simulink subsystem "fluxObserver"  (R2023b)
settings: Solver=VariableStepAuto  StartTime=0.0  StopTime=10.0  RelTol=1e-3
values from neighbouring files (symbols this model uses):
  motor = setMotorParameters("SynRelLaplace")    [initSimulinkObs.m]    (also in setMotorParameters.m = struct)
  Ts = 1e-4    (= 0.0001)    [initSimulinkObs.m]
undefined symbols (not defined in the file or in its folder): DiscIntNeverNeededParam, math, observer
settings Model: Creator=rdelpoux  LastModifiedBy=rdelpoux
settings ModelReferenceCC: UpdateModelReferenceTargets=IfOutOfDate
settings RTWCC: GPUComputeCapability=5.0
settings ConfigComp: CovBoundaryAbsTol=1.0e-5

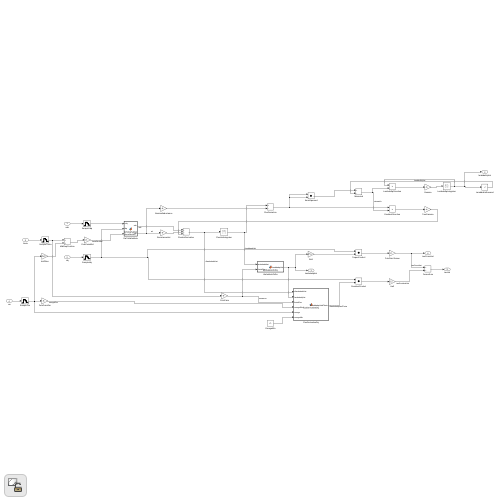
[thumbnail: Simulink's stored preview of the top-level diagram]
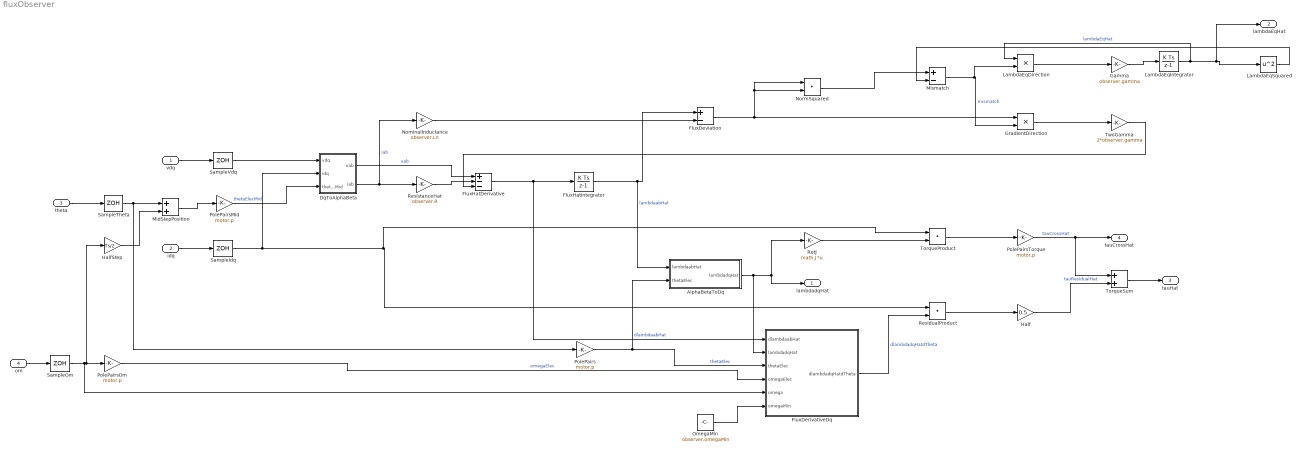
== system fluxObserver ==
  vdq : Inport
  idq : Inport  Port=2
  theta : Inport  Port=3
  om : Inport  Port=4
  AlphaBetaToDq : MATLAB Function  TreatAsAtomicUnit=on
  DqToAlphaBeta : MATLAB Function  TreatAsAtomicUnit=on
  FluxDerivativeDq : MATLAB Function  TreatAsAtomicUnit=on
  FluxDeviation : Sum  Inputs=+-
  FluxHatDerivative : Sum  Inputs=+--
  FluxHatIntegrator : DiscreteIntegrator  InitialCondition=observer.lambda0  SampleTime=Ts  ICPrevOutput=DiscIntNeverNeededParam  ICPrevScaledInput=DiscIntNeverNeededParam
  Gamma : Gain  Gain=observer.gamma
  GradientDirection : Product
  Half : Gain  Gain=0.5
  HalfStep : Gain  Gain=Ts/2
  LambdaEqDirection : Product
  LambdaEqIntegrator : DiscreteIntegrator  InitialCondition=observer.lambdaEq0  SampleTime=Ts  ICPrevOutput=DiscIntNeverNeededParam  ICPrevScaledInput=DiscIntNeverNeededParam
  LambdaEqSquared : Math  Operator=square
  MidStepPosition : Sum
  Mismatch : Sum  Inputs=+-
  NominalInductance : Gain  Gain=observer.Ln
  NormSquared : DotProduct  OutDataTypeStr=Inherit: Inherit via internal rule
  OmegaMin : Constant  Value=observer.omegaMin
  PolePairs : Gain  Gain=motor.p
  PolePairsMid : Gain  Gain=motor.p
  PolePairsOm : Gain  Gain=motor.p
  PolePairsTorque : Gain  Gain=motor.p
  ResidualProduct : DotProduct  OutDataTypeStr=Inherit: Inherit via internal rule
  ResistanceHat : Gain  Gain=observer.R
  RotJ : Gain  Gain=math.J  Multiplication=Matrix(K*u)
  SampleIdq : ZeroOrderHold  SampleTime=Ts
  SampleOm : ZeroOrderHold  SampleTime=Ts
  SampleTheta : ZeroOrderHold  SampleTime=Ts
  SampleVdq : ZeroOrderHold  SampleTime=Ts
  TorqueProduct : DotProduct  OutDataTypeStr=Inherit: Inherit via internal rule
  TorqueSum : Sum
  TwoGamma : Gain  Gain=2*observer.gamma
  lambdadqHat : Outport
  lambdaEqHat : Outport  Port=2
  tauHat : Outport  Port=3
  tauCrossHat : Outport  Port=4
  wires:
  PolePairsMid/1 -> DqToAlphaBeta/3(thetaElecMid)  "thetaElecMid"
  MidStepPosition/1 -> PolePairsMid/1
  HalfStep/1 -> MidStepPosition/2
  ResidualProduct/1 -> Half/1
  TorqueSum/1 -> tauHat/1
  Half/1 -> TorqueSum/2  "tauResidualHat"
  PolePairsTorque/1 -> tauCrossHat/1, TorqueSum/1  "tauCrossHat"
  SampleOm/1 -> FluxDerivativeDq/5(omega), HalfStep/1, PolePairsOm/1
  om/1 -> SampleOm/1
  AlphaBetaToDq/1(lambdadqHat) -> FluxDerivativeDq/2(lambdadqHat), RotJ/1, lambdadqHat/1
  TorqueProduct/1 -> PolePairsTorque/1
  RotJ/1 -> TorqueProduct/2
  Gamma/1 -> LambdaEqIntegrator/1
  LambdaEqDirection/1 -> Gamma/1
  FluxHatDerivative/1 -> FluxHatIntegrator/1, FluxDerivativeDq/1(dlambdaabHat)  "dlambdaabHat"
  TwoGamma/1 -> FluxHatDerivative/3
  ResistanceHat/1 -> FluxHatDerivative/2
  DqToAlphaBeta/1(vab) -> FluxHatDerivative/1  "vab"
  GradientDirection/1 -> TwoGamma/1
  Mismatch/1 -> LambdaEqDirection/2, GradientDirection/2  "mismatch"
  LambdaEqSquared/1 -> Mismatch/2
  NormSquared/1 -> Mismatch/1
  LambdaEqIntegrator/1 -> LambdaEqDirection/1, lambdaEqHat/1, LambdaEqSquared/1  "lambdaEqHat"
  FluxDeviation/1 -> GradientDirection/1, NormSquared/2, NormSquared/1
  NominalInductance/1 -> FluxDeviation/2
  FluxHatIntegrator/1 -> FluxDeviation/1, AlphaBetaToDq/1(lambdaabHat)  "lambdaabHat"
  SampleVdq/1 -> DqToAlphaBeta/1(vdq)
  SampleTheta/1 -> MidStepPosition/1, PolePairs/1
  theta/1 -> SampleTheta/1
  idq/1 -> SampleIdq/1
  vdq/1 -> SampleVdq/1
  SampleIdq/1 -> DqToAlphaBeta/2(idq), TorqueProduct/1, ResidualProduct/1
  PolePairs/1 -> AlphaBetaToDq/2(thetaElec), FluxDerivativeDq/3(thetaElec)  "thetaElec"
  DqToAlphaBeta/2(iab) -> NominalInductance/1, ResistanceHat/1  "iab"
  PolePairsOm/1 -> FluxDerivativeDq/4(omegaElec)  "omegaElec"
  OmegaMin/1 -> FluxDerivativeDq/6(omegaMin)
  FluxDerivativeDq/1(dlambdadqHatdTheta) -> ResidualProduct/2  "dlambdadqHatdTheta"

== matlab function fluxObserver/AlphaBetaToDq ==
  data: lambdaabHat input size=2; lambdadqHat output size=2; thetaElec input
function lambdadqHat = alphaBetaToDq(lambdaabHat, thetaElec)
%ALPHABETATODQ Passage du repere alphabeta au repere dq : x_dq = P(p*theta)' x_ab.
c = cos(thetaElec);
s = sin(thetaElec);
P = [c, -s; s, c];
lambdadqHat = P' * lambdaabHat(:);
end

== matlab function fluxObserver/DqToAlphaBeta ==
  data: vdq input size=2; vab output size=2; idq input size=2; thetaElecMid input; iab output size=2
function [vab, iab] = dqToAlphaBeta(vdq, idq, thetaElecMid)
%DQTOALPHABETA Passage du repere dq au repere alphabeta : x_ab = P(p*theta)' x_dq.
%   Convention coherente avec le modele (d(lambda_dq)/dt = ... - p*w*J*lambda_dq).
%   L'angle est pris a mi-pas (theta + w*Ts/2) : c'est la valeur moyenne de la
%   rotation sur le pas d'integration, ce qui supprime le retard d'un demi-pas
%   de l'integration d'Euler explicite sur des grandeurs tournantes.
c = cos(thetaElecMid);
s = sin(thetaElecMid);
P = [c, -s; s, c];
vab = P * vdq(:);
iab = P * idq(:);
end

== matlab function fluxObserver/FluxDerivativeDq ==
  data: dlambdaabHat input size=2; dlambdadqHatdTheta output size=2; lambdadqHat input size=2; thetaElec input; omegaElec input; omega input; omegaMin input
function dlambdadqHatdTheta = fluxDerivativeDq(dlambdaabHat, lambdadqHat, thetaElec, omegaElec, omega, omegaMin)
%FLUXDERIVATIVEDQ Derivee du flux estime dq par rapport a la position mecanique.
%   Avec lambda_dq = P(p*theta) lambda_ab et P dP'/d(p*theta) = J (eq. 31) :
%     d(lambda_dq)/dt = P d(lambda_ab)/dt - p*omega*J*lambda_dq
%   puis d(lambda_dq)/dtheta = d(lambda_dq)/dt / omega, |omega| borne par omegaMin.
c = cos(thetaElec);
s = sin(thetaElec);
P = [c, s; -s, c];
J = [0, -1; 1, 0];
dlambdadqHatdt = P * dlambdaabHat(:) - omegaElec * (J * lambdadqHat(:));
if omega >= 0
    omegaSafe = max(omega, omegaMin);
else
    omegaSafe = min(omega, -omegaMin);
end
dlambdadqHatdTheta = dlambdadqHatdt / omegaSafe;
end
